simulink model "Drone"  (R2026a)
settings: Solver=VariableStepAuto  StopTime=500
undefined symbols (not defined in the file): magnitude
libraries: slpidlib x4, simulink_extras x1, sl3dlib x1, sim3dlib x1, uavsim3dlib x1
settings Model: Creator=siddharthreddy  LastModifiedBy=Sid

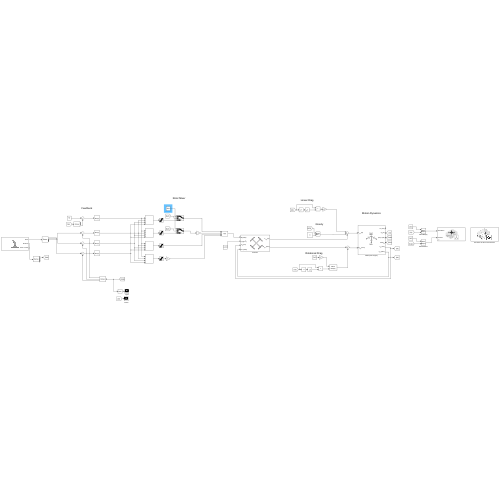
[thumbnail: Simulink's stored preview of the top-level diagram]
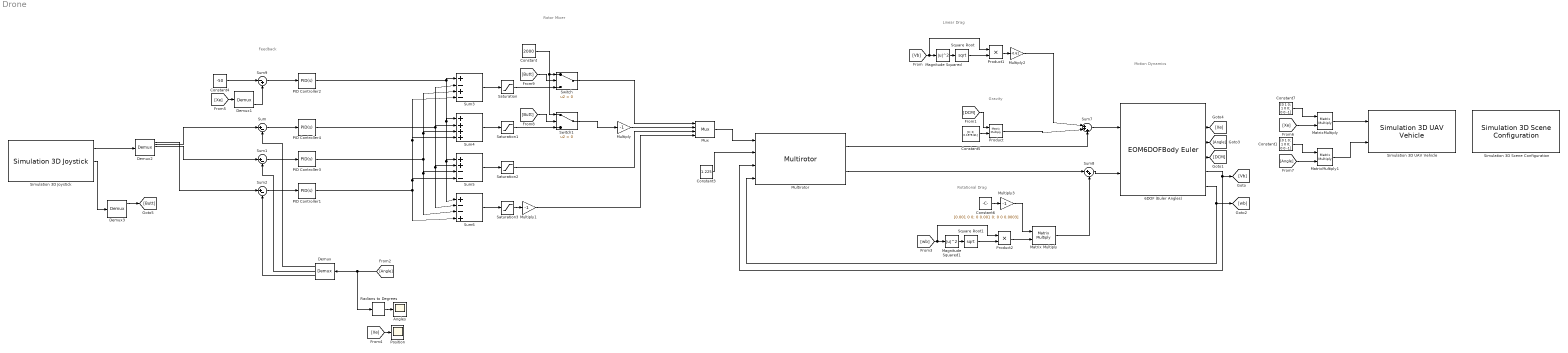
== system Drone ==
  note: Motion Dynamics
  note: Rotor Mixer
  note: Feedback
  note: Gravity
  note: Linear Drag
  note: Rotational Drag
  6DOF (Euler Angles) : EOM6DOFBodyEuler  xme_0=[0 0 -40]  eul_0=[.25 .25 .5]  mass_0=0.15  inertia=[0.0003 0 0; 0 0.0003 0; 0 0 0.0003]
  Angles : Scope
      settings: ActiveDisplayYMinimum=-79.706832912705636  ActiveDisplayYMaximum=125.45902835260904
  Constant : Constant  Value=2000
  Constant1 : Constant  Value=[0 1 0; 1 0 0; 0 0 -1]
  Constant3 : Constant  Value=1.225
  Constant4 : Constant  Value=-50
  Constant5 : Constant  Value=[0; 0; 0.15*9.81]
  Constant6 : Constant  Value=[0.001 0 0; 0 0.001 0; 0 0 0.0003]
  Constant7 : Constant  Value=[0 1 0; 1 0 0; 0 0 -1]
  Demux : Demux  Outputs=3
      settings: DisplayOption=none
  Demux1 : Demux  Outputs=3
      settings: DisplayOption=none
  Demux2 : Demux  Outputs=6
      settings: DisplayOption=none
  Demux3 : Demux  Outputs=8
      settings: DisplayOption=none
  Magnitude Squared : Math  Operator=magnitude^2
  Magnitude Squared1 : Math  Operator=magnitude^2
  Matrix Multiply : Product  Multiplication=Matrix(*)
  MatrixMultiply : Product  Multiplication=Matrix(*)
  MatrixMultiply1 : Product  Multiplication=Matrix(*)
  Multiply : Gain  Gain=-1
  Multiply1 : Gain  Gain=-1
  Multiply2 : Gain  Gain=-0.61
  Multiply3 : Gain  Gain=-1
  Multirotor : Multirotor  modelMode=With flap effects  armLength=0.06  rotorHeight=0  CT=0.08  CQ=0.001  radius=0.065/2
  Mux : Mux
  PID Controller1 : slpidlib/PID Controller  Controller=PID  Form=Parallel  TimeDomain=Continuous-time  UseExternalTs=off  SampleTime=-1  IntegratorMethod=Forward Euler  FilterMethod=Forward Euler  ControllerParametersSource=internal  P=1421.28268044684  I=470.589569781493  UseKiTs=off  D=956.469408662535  UseExternalDerivativeSource=off  N=11.7175649403718  UseFilter=on  TunerSelectOption=Transfer Function Based (PID Tuner App)  InitialConditionSource=internal  InitialConditionForIntegrator=0  InitialConditionForFilter=0  DifferentiatorICPrevScaledInput=0  ExternalReset=none  TrackingMode=off  Kt=1  LimitOutput=off  SatLimitsSource=internal  UpperSaturationLimit=inf  LowerSaturationLimit=-inf  LinearizeAsGain=on  AntiWindupMode=none  Kb=1  LimitIntegrator=off  UpperIntegratorSaturationLimit=inf  LowerIntegratorSaturationLimit=-inf  POutMin=[]  POutMax=[]  IOutMin=[]  IOutMax=[]  DOutMin=[]  DOutMax=[]  NOutMin=[]  NOutMax=[]  SumOutMin=[]  SumOutMax=[]  SaturationOutMin=[]  SaturationOutMax=[]  PParamMin=[]  PParamMax=[]  IParamMin=[]  IParamMax=[]  DParamMin=[]  DParamMax=[]  NParamMin=[]  NParamMax=[]  KbParamMin=[]  KbParamMax=[]  KtParamMin=[]  KtParamMax=[]  KbOutMin=[]  KbOutMax=[]  KtOutMin=[]  KtOutMax=[]  IntegratorOutMin=[]  IntegratorOutMax=[]  FilterOutMin=[]  FilterOutMax=[]  SumI1OutMin=[]  SumI1OutMax=[]  SumI2OutMin=[]  SumI2OutMax=[]  SumI3OutMin=[]  SumI3OutMax=[]  SumI4OutMin=[]  SumI4OutMax=[]  SumDOutMin=[]  SumDOutMax=[]  DifferentiatorOutMin=[]  DifferentiatorOutMax=[]  FilterDiffOutCoefMin=[]  FilterDiffOutCoefMax=[]  ReciprocalOutMin=[]  ReciprocalOutMax=[]  SumDenOutMin=[]  SumDenOutMax=[]  SumNumOutMin=[]  SumNumOutMax=[]  DivideOutMin=[]  DivideOutMax=[]  UdiffTsProdOutMin=[]  UdiffTsProdOutMax=[]  NTsProdOutMin=[]  NTsProdOutMax=[]  UintegralTsProdOutMin=[]  UintegralTsProdOutMax=[]  UngainTsProdOutMin=[]  UngainTsProdOutMax=[]  ClampingZeroOutDataTypeStr=Inherit: Inherit via back propagation  ClampingZeroOutMin=[]  ClampingZeroOutMax=[]  FilterDenConstantOutDataTypeStr=Inherit: Inherit via back propagation  FilterDenConstantOutMin=[]  FilterDenConstantOutMax=[]  PCopyOutDataTypeStr=Inherit: Inherit via back propagation  PCopyOutMin=[]  PCopyOutMax=[]  NCopyOutDataTypeStr=Inherit: Inherit via back propagation  NCopyOutMin=[]  NCopyOutMax=[]  IntegratorContinuousStateAttributes=''  IntegratorStateMustResolveToSignalObject=off  IntegratorRTWStateStorageClass=Auto  FilterContinuousStateAttributes=''  FilterStateMustResolveToSignalObject=off  FilterRTWStateStorageClass=Auto  ParallelPVariant=InternalParameters  IdealPVariant=Disabled  IVariant=InternalParameters  DVariant=InternalParameters  IntegratorVariant=Continuous  SatVariant=Disabled  AWVariant=Passthrough  PCopyVariant=Disabled  TRVariant=Disabled  FdbkBlocksVariant=Forward  IdealPFdbkVariant=Disabled  SatFdbkVariant=Disabled  DerivativeFilterVariant=ContFilter  NVariant=InternalParameters  NCopyVariant=Disabled  FilterICVariant=InternalICsFilter  IntegratorICVariant=InternalICs  ExternalResetVariant=Disabled  TRSumVariant=Passthrough  SumFdbkVariant=Disabled  SumVariant=Sum_PID  TsampFilterVariant=InternalTs  TsampNgainVariant=Passthrough  TsampIntegralVariant=Disabled_SignalSpec  ExternalSaturationOutDataTypeStr=Inherit: Same as second input  DerivativeSourceVariant=ErrorSignal  PreIntVariant=InternalPreInt
  PID Controller2 : slpidlib/PID Controller  Controller=PID  Form=Parallel  TimeDomain=Continuous-time  UseExternalTs=off  SampleTime=-1  IntegratorMethod=Forward Euler  FilterMethod=Forward Euler  ControllerParametersSource=internal  P=465.549469406637  I=214.212668672937  UseKiTs=off  D=189.884905448547  UseExternalDerivativeSource=off  N=1142.8279760416  UseFilter=on  TunerSelectOption=Transfer Function Based (PID Tuner App)  InitialConditionSource=internal  InitialConditionForIntegrator=0  InitialConditionForFilter=0  DifferentiatorICPrevScaledInput=0  ExternalReset=none  TrackingMode=off  Kt=1  LimitOutput=off  SatLimitsSource=internal  UpperSaturationLimit=inf  LowerSaturationLimit=-inf  LinearizeAsGain=on  AntiWindupMode=none  Kb=1  LimitIntegrator=off  UpperIntegratorSaturationLimit=inf  LowerIntegratorSaturationLimit=-inf  POutMin=[]  POutMax=[]  IOutMin=[]  IOutMax=[]  DOutMin=[]  DOutMax=[]  NOutMin=[]  NOutMax=[]  SumOutMin=[]  SumOutMax=[]  SaturationOutMin=[]  SaturationOutMax=[]  PParamMin=[]  PParamMax=[]  IParamMin=[]  IParamMax=[]  DParamMin=[]  DParamMax=[]  NParamMin=[]  NParamMax=[]  KbParamMin=[]  KbParamMax=[]  KtParamMin=[]  KtParamMax=[]  KbOutMin=[]  KbOutMax=[]  KtOutMin=[]  KtOutMax=[]  IntegratorOutMin=[]  IntegratorOutMax=[]  FilterOutMin=[]  FilterOutMax=[]  SumI1OutMin=[]  SumI1OutMax=[]  SumI2OutMin=[]  SumI2OutMax=[]  SumI3OutMin=[]  SumI3OutMax=[]  SumI4OutMin=[]  SumI4OutMax=[]  SumDOutMin=[]  SumDOutMax=[]  DifferentiatorOutMin=[]  DifferentiatorOutMax=[]  FilterDiffOutCoefMin=[]  FilterDiffOutCoefMax=[]  ReciprocalOutMin=[]  ReciprocalOutMax=[]  SumDenOutMin=[]  SumDenOutMax=[]  SumNumOutMin=[]  SumNumOutMax=[]  DivideOutMin=[]  DivideOutMax=[]  UdiffTsProdOutMin=[]  UdiffTsProdOutMax=[]  NTsProdOutMin=[]  NTsProdOutMax=[]  UintegralTsProdOutMin=[]  UintegralTsProdOutMax=[]  UngainTsProdOutMin=[]  UngainTsProdOutMax=[]  ClampingZeroOutDataTypeStr=Inherit: Inherit via back propagation  ClampingZeroOutMin=[]  ClampingZeroOutMax=[]  FilterDenConstantOutDataTypeStr=Inherit: Inherit via back propagation  FilterDenConstantOutMin=[]  FilterDenConstantOutMax=[]  PCopyOutDataTypeStr=Inherit: Inherit via back propagation  PCopyOutMin=[]  PCopyOutMax=[]  NCopyOutDataTypeStr=Inherit: Inherit via back propagation  NCopyOutMin=[]  NCopyOutMax=[]  IntegratorContinuousStateAttributes=''  IntegratorStateMustResolveToSignalObject=off  IntegratorRTWStateStorageClass=Auto  FilterContinuousStateAttributes=''  FilterStateMustResolveToSignalObject=off  FilterRTWStateStorageClass=Auto  ParallelPVariant=InternalParameters  IdealPVariant=Disabled  IVariant=InternalParameters  DVariant=InternalParameters  IntegratorVariant=Continuous  SatVariant=Disabled  AWVariant=Passthrough  PCopyVariant=Disabled  TRVariant=Disabled  FdbkBlocksVariant=Forward  IdealPFdbkVariant=Disabled  SatFdbkVariant=Disabled  DerivativeFilterVariant=ContFilter  NVariant=InternalParameters  NCopyVariant=Disabled  FilterICVariant=InternalICsFilter  IntegratorICVariant=InternalICs  ExternalResetVariant=Disabled  TRSumVariant=Passthrough  SumFdbkVariant=Disabled  SumVariant=Sum_PID  TsampFilterVariant=InternalTs  TsampNgainVariant=Passthrough  TsampIntegralVariant=Disabled_SignalSpec  ExternalSaturationOutDataTypeStr=Inherit: Same as second input  DerivativeSourceVariant=ErrorSignal  PreIntVariant=InternalPreInt
  PID Controller3 : slpidlib/PID Controller  Controller=PID  Form=Parallel  TimeDomain=Continuous-time  UseExternalTs=off  SampleTime=-1  IntegratorMethod=Forward Euler  FilterMethod=Forward Euler  ControllerParametersSource=internal  P=1.53294785605493  I=0.217782758826352  UseKiTs=off  D=2.68640511728312  UseExternalDerivativeSource=off  N=361.393937805181  UseFilter=on  TunerSelectOption=Transfer Function Based (PID Tuner App)  InitialConditionSource=internal  InitialConditionForIntegrator=0  InitialConditionForFilter=0  DifferentiatorICPrevScaledInput=0  ExternalReset=none  TrackingMode=off  Kt=1  LimitOutput=off  SatLimitsSource=internal  UpperSaturationLimit=inf  LowerSaturationLimit=-inf  LinearizeAsGain=on  AntiWindupMode=none  Kb=1  LimitIntegrator=off  UpperIntegratorSaturationLimit=inf  LowerIntegratorSaturationLimit=-inf  POutMin=[]  POutMax=[]  IOutMin=[]  IOutMax=[]  DOutMin=[]  DOutMax=[]  NOutMin=[]  NOutMax=[]  SumOutMin=[]  SumOutMax=[]  SaturationOutMin=[]  SaturationOutMax=[]  PParamMin=[]  PParamMax=[]  IParamMin=[]  IParamMax=[]  DParamMin=[]  DParamMax=[]  NParamMin=[]  NParamMax=[]  KbParamMin=[]  KbParamMax=[]  KtParamMin=[]  KtParamMax=[]  KbOutMin=[]  KbOutMax=[]  KtOutMin=[]  KtOutMax=[]  IntegratorOutMin=[]  IntegratorOutMax=[]  FilterOutMin=[]  FilterOutMax=[]  SumI1OutMin=[]  SumI1OutMax=[]  SumI2OutMin=[]  SumI2OutMax=[]  SumI3OutMin=[]  SumI3OutMax=[]  SumI4OutMin=[]  SumI4OutMax=[]  SumDOutMin=[]  SumDOutMax=[]  DifferentiatorOutMin=[]  DifferentiatorOutMax=[]  FilterDiffOutCoefMin=[]  FilterDiffOutCoefMax=[]  ReciprocalOutMin=[]  ReciprocalOutMax=[]  SumDenOutMin=[]  SumDenOutMax=[]  SumNumOutMin=[]  SumNumOutMax=[]  DivideOutMin=[]  DivideOutMax=[]  UdiffTsProdOutMin=[]  UdiffTsProdOutMax=[]  NTsProdOutMin=[]  NTsProdOutMax=[]  UintegralTsProdOutMin=[]  UintegralTsProdOutMax=[]  UngainTsProdOutMin=[]  UngainTsProdOutMax=[]  ClampingZeroOutDataTypeStr=Inherit: Inherit via back propagation  ClampingZeroOutMin=[]  ClampingZeroOutMax=[]  FilterDenConstantOutDataTypeStr=Inherit: Inherit via back propagation  FilterDenConstantOutMin=[]  FilterDenConstantOutMax=[]  PCopyOutDataTypeStr=Inherit: Inherit via back propagation  PCopyOutMin=[]  PCopyOutMax=[]  NCopyOutDataTypeStr=Inherit: Inherit via back propagation  NCopyOutMin=[]  NCopyOutMax=[]  IntegratorContinuousStateAttributes=''  IntegratorStateMustResolveToSignalObject=off  IntegratorRTWStateStorageClass=Auto  FilterContinuousStateAttributes=''  FilterStateMustResolveToSignalObject=off  FilterRTWStateStorageClass=Auto  ParallelPVariant=InternalParameters  IdealPVariant=Disabled  IVariant=InternalParameters  DVariant=InternalParameters  IntegratorVariant=Continuous  SatVariant=Disabled  AWVariant=Passthrough  PCopyVariant=Disabled  TRVariant=Disabled  FdbkBlocksVariant=Forward  IdealPFdbkVariant=Disabled  SatFdbkVariant=Disabled  DerivativeFilterVariant=ContFilter  NVariant=InternalParameters  NCopyVariant=Disabled  FilterICVariant=InternalICsFilter  IntegratorICVariant=InternalICs  ExternalResetVariant=Disabled  TRSumVariant=Passthrough  SumFdbkVariant=Disabled  SumVariant=Sum_PID  TsampFilterVariant=InternalTs  TsampNgainVariant=Passthrough  TsampIntegralVariant=Disabled_SignalSpec  ExternalSaturationOutDataTypeStr=Inherit: Same as second input  DerivativeSourceVariant=ErrorSignal  PreIntVariant=InternalPreInt
  PID Controller4 : slpidlib/PID Controller  Controller=PID  Form=Parallel  TimeDomain=Continuous-time  UseExternalTs=off  SampleTime=-1  IntegratorMethod=Forward Euler  FilterMethod=Forward Euler  ControllerParametersSource=internal  P=-1.53294785605493  I=-0.217782758826352  UseKiTs=off  D=-2.68640511728312  UseExternalDerivativeSource=off  N=361.393937805181  UseFilter=on  TunerSelectOption=Transfer Function Based (PID Tuner App)  InitialConditionSource=internal  InitialConditionForIntegrator=0  InitialConditionForFilter=0  DifferentiatorICPrevScaledInput=0  ExternalReset=none  TrackingMode=off  Kt=1  LimitOutput=off  SatLimitsSource=internal  UpperSaturationLimit=inf  LowerSaturationLimit=-inf  LinearizeAsGain=on  AntiWindupMode=none  Kb=1  LimitIntegrator=off  UpperIntegratorSaturationLimit=inf  LowerIntegratorSaturationLimit=-inf  POutMin=[]  POutMax=[]  IOutMin=[]  IOutMax=[]  DOutMin=[]  DOutMax=[]  NOutMin=[]  NOutMax=[]  SumOutMin=[]  SumOutMax=[]  SaturationOutMin=[]  SaturationOutMax=[]  PParamMin=[]  PParamMax=[]  IParamMin=[]  IParamMax=[]  DParamMin=[]  DParamMax=[]  NParamMin=[]  NParamMax=[]  KbParamMin=[]  KbParamMax=[]  KtParamMin=[]  KtParamMax=[]  KbOutMin=[]  KbOutMax=[]  KtOutMin=[]  KtOutMax=[]  IntegratorOutMin=[]  IntegratorOutMax=[]  FilterOutMin=[]  FilterOutMax=[]  SumI1OutMin=[]  SumI1OutMax=[]  SumI2OutMin=[]  SumI2OutMax=[]  SumI3OutMin=[]  SumI3OutMax=[]  SumI4OutMin=[]  SumI4OutMax=[]  SumDOutMin=[]  SumDOutMax=[]  DifferentiatorOutMin=[]  DifferentiatorOutMax=[]  FilterDiffOutCoefMin=[]  FilterDiffOutCoefMax=[]  ReciprocalOutMin=[]  ReciprocalOutMax=[]  SumDenOutMin=[]  SumDenOutMax=[]  SumNumOutMin=[]  SumNumOutMax=[]  DivideOutMin=[]  DivideOutMax=[]  UdiffTsProdOutMin=[]  UdiffTsProdOutMax=[]  NTsProdOutMin=[]  NTsProdOutMax=[]  UintegralTsProdOutMin=[]  UintegralTsProdOutMax=[]  UngainTsProdOutMin=[]  UngainTsProdOutMax=[]  ClampingZeroOutDataTypeStr=Inherit: Inherit via back propagation  ClampingZeroOutMin=[]  ClampingZeroOutMax=[]  FilterDenConstantOutDataTypeStr=Inherit: Inherit via back propagation  FilterDenConstantOutMin=[]  FilterDenConstantOutMax=[]  PCopyOutDataTypeStr=Inherit: Inherit via back propagation  PCopyOutMin=[]  PCopyOutMax=[]  NCopyOutDataTypeStr=Inherit: Inherit via back propagation  NCopyOutMin=[]  NCopyOutMax=[]  IntegratorContinuousStateAttributes=''  IntegratorStateMustResolveToSignalObject=off  IntegratorRTWStateStorageClass=Auto  FilterContinuousStateAttributes=''  FilterStateMustResolveToSignalObject=off  FilterRTWStateStorageClass=Auto  ParallelPVariant=InternalParameters  IdealPVariant=Disabled  IVariant=InternalParameters  DVariant=InternalParameters  IntegratorVariant=Continuous  SatVariant=Disabled  AWVariant=Passthrough  PCopyVariant=Disabled  TRVariant=Disabled  FdbkBlocksVariant=Forward  IdealPFdbkVariant=Disabled  SatFdbkVariant=Disabled  DerivativeFilterVariant=ContFilter  NVariant=InternalParameters  NCopyVariant=Disabled  FilterICVariant=InternalICsFilter  IntegratorICVariant=InternalICs  ExternalResetVariant=Disabled  TRSumVariant=Passthrough  SumFdbkVariant=Disabled  SumVariant=Sum_PID  TsampFilterVariant=InternalTs  TsampNgainVariant=Passthrough  TsampIntegralVariant=Disabled_SignalSpec  ExternalSaturationOutDataTypeStr=Inherit: Same as second input  DerivativeSourceVariant=ErrorSignal  PreIntVariant=InternalPreInt
  Position : Scope
      settings: ActiveDisplayYMinimum=-335.35566969073909  ActiveDisplayYMaximum=208.27591374665826
  Product : Product  Multiplication=Matrix(*)
  Product1 : Product
  Product2 : Product
  Radians to Degrees : simulink_extras/Transformations/Radians to Degrees
  Saturation{,1..3} (4 alike) : Saturate  UpperLimit=3000  LowerLimit=0
  Simulation 3D Joystick : sl3dlib/Simulation 3D/Hardware Interface/Simulation 3D Joystick  joyid=1  adjustports=on  forcefeed=off
  Simulation 3D Scene Configuration : sim3dlib/Simulation 3D Scene Configuration  Priority=0  ProjectFormat=Default Scenes  SceneDesc=US city block  ProjectName=C:\Program Files\MATLAB\R2026a\toolbox\shared\sim3d_projects\automotive_project_windows\UE\WindowsNoEditor\VehicleSimulation.exe  ScenePath=/Game/Maps/USCityBlock  EnableOpenDRIVE=off  vehTagList={'Custom';'Scene Origin';'SimulinkVehicle1'}  vehTag=SimulinkVehicle1  AttachedCameraRelativeTranslation=[0 0 0]  FreeCameraDefaultInitialTranslation=[-6, 0, 2]  AttachedCameraRelativeRotation=[0, -15, 0]  FreeCameraDefaultInitialRotation=[0, -15, 0]  ViewpointName=Custom  FreeCameraInitialTranslation=[0, 0, 0]  FreeCameraInitialRotation=[0, 0, 0]  OpVisEn=off  Ts=1/60  EnableWindow=on  EnableRemoteAccess=off  SimulationMode=CoSimulation  SimulateUsing=Interpreted execution  EnableAnimationRecording=off  OverrideDefaultRecording=off  AnimationRecordingFileName=sim3dAnimation.mat  AnimationRecordingInterval=[0 inf]  EnableWeather=off  SunAzimuth=90  SunAltitude=40.0  EnableGeospatialSun=off  Latitude=0  Longitude=0  Date=2023-01-01  Time=10:30:00  GeoTimeZone=-5.0  SunDaylightSaving=off  wind=1  clouds=10  EnableVolumetricClouds=off  CloudCoverage=0  CloudAltitude=6  fog=0  rain=0  RaindropsEffect=off  SnowDensity=0  EnableGeospatial=off  TilesetSource=Earth terrain  UseTrueOrigin=off  OriginHeight=200  OriginLatitude=40.744652  OriginLongitude=-73.988864  MapStyle=Aerial  AdditionalAssetIDs=[]  UseAdvancedSunSky=off  SolarTime=11  TimeZone=-5  Day=21  Month=9  Year=2022  UseDaylightSavingTime=on  DSTStartDay=10  DSTStartMonth=3  DSTEndDay=3  DSTEndMonth=11  DSTSwitchHour=2  sensorTag=MainCamera1  sensorId=1  sensorName=MainCamera1  mountLoc=Origin  offsetFlag=off  tmountOffset=[0, 0, 0]  rmountOffset=[0, 0, 0]  HorizontalResolution=1280  VerticalResolution=720  HorizontalFOV=60  mountPoint=[0 0 0]  mountOrientation=[0 0 0]  aMode=4  ID=1  GeoTrigger=Inactive  ViewNameList={'Custom'}  ViewTranslationList={'[0 0 0]'}  ViewRotationList={'[0 0 0]'}
      settings: LibrarySourceBlock=uavsim3dlib/Simulation 3D Scene Configuration
  Simulation 3D UAV Vehicle : uavsim3dlib/Simulation 3D UAV Vehicle  Priority=-1  Mesh=Quadrotor  MeshPath=/MathWorksUAVContent/UAVs/HexaRotorUAV/HexaRotor.HexaRotor  Color=Black  ActorName=SimulinkVehicle1  UseGlobalFrame=off  InitialTranslation=[0 0 0]  InitialRotation=[0 0 0]  InitialTranslationGlobal=[0 0 0]  InitialGeoOrigin=[0 0 0]  InitialRotationGlobal=[0 0 0]  SampleTime=-1  ActorType=SimulinkVehicle  ID=1  aMode=4  ActorTag=SimulinkVehicle1
  Square Root : Sqrt
  Square Root1 : Sqrt
  Sum : Sum  Inputs=|+-
  Sum1 : Sum  Inputs=|+-
  Sum2 : Sum  Inputs=|+-
  Sum3 : Sum  Inputs=|+-+-
  Sum4 : Sum  Inputs=|++++
  Sum5 : Sum  Inputs=|++--
  Sum6 : Sum  Inputs=|+--+
  Sum7 : Sum  Inputs=|+++
  Sum8 : Sum  Inputs=|++
  Sum9 : Sum  Inputs=|-+
  Switch : Switch  Criteria=u2 > Threshold  SaturateOnIntegerOverflow=off  InputSameDT=off
  Switch1 : Switch  Criteria=u2 > Threshold  SaturateOnIntegerOverflow=off  InputSameDT=off
  wires:
  Sum/1 -> PID Controller4/1
  Sum2/1 -> PID Controller1/1
  Demux/1 -> Sum/2
  Demux/2 -> Sum1/2
  Demux/3 -> Sum2/2
  PID Controller1/1 -> Sum6/4, Sum3/4, Sum4/4, Sum5/4
  PID Controller3/1 -> Sum6/3, Sum5/3, Sum3/3, Sum4/3
  PID Controller4/1 -> Sum3/2, Sum4/2, Sum6/2, Sum5/2
  Mux/1 -> Multirotor/1
  Constant3/1 -> Multirotor/2
  PID Controller2/1 -> Sum4/1, Sum5/1, Sum6/1, Sum3/1
  Sum1/1 -> PID Controller3/1
  Sum3/1 -> Saturation/1
  Sum4/1 -> Saturation1/1
  Sum5/1 -> Saturation2/1
  Sum6/1 -> Saturation3/1
  Radians to Degrees/1 -> Angles/1
  Saturation2/1 -> Mux/3
  Saturation3/1 -> Multiply1/1
  Multiply/1 -> Mux/2
  Multiply1/1 -> Mux/4
  Magnitude Squared/1 -> Square Root/1
  Product1/1 -> Multiply2/1
  [Vb] -> Product1/1, Magnitude Squared/1
  6DOF (Euler Angles)/4 -> [DCM]
  Square Root/1 -> Product1/2
  6DOF (Euler Angles)/5 -> [Vb], Multirotor/3
  6DOF (Euler Angles)/6 -> [wb], Multirotor/4
  [DCM] -> Product/1
  Constant5/1 -> Product/2
  Multirotor/1 -> Sum7/3
  Multiply2/1 -> Sum7/1
  Sum7/1 -> 6DOF (Euler Angles)/1
  6DOF (Euler Angles)/3 -> [Angle]
  [Angle] -> Radians to Degrees/1, Demux/1
  Product/1 -> Sum7/2
  Product2/1 -> Matrix Multiply/2
  [wb] -> Product2/1, Magnitude Squared1/1
  Magnitude Squared1/1 -> Square Root1/1
  Square Root1/1 -> Product2/2
  Constant6/1 -> Multiply3/1
  Multiply3/1 -> Matrix Multiply/1
  Matrix Multiply/1 -> Sum8/2
  Sum8/1 -> 6DOF (Euler Angles)/2
  Multirotor/2 -> Sum8/1
  6DOF (Euler Angles)/2 -> [Xe]
  [Xe] -> Position/1
  Constant4/1 -> Sum9/1
  Sum9/1 -> PID Controller2/1
  Demux1/3 -> Sum9/2
  [Xe] -> Demux1/1
  Constant7/1 -> MatrixMultiply/1
  [Xe] -> MatrixMultiply/2
  MatrixMultiply/1 -> Simulation 3D UAV Vehicle/1
  Simulation 3D Joystick/1 -> Demux2/1
  [Angle] -> MatrixMultiply1/2
  Constant1/1 -> MatrixMultiply1/1
  MatrixMultiply1/1 -> Simulation 3D UAV Vehicle/2
  Simulation 3D Joystick/2 -> Demux3/1
  Demux2/2 -> Sum/1
  Demux2/3 -> Sum1/1
  Demux2/1 -> Sum2/1
  Switch/1 -> Mux/1
  Switch1/1 -> Multiply/1
  Saturation/1 -> Switch/3
  Saturation1/1 -> Switch1/3
  [Butt] -> Switch/2
  [Butt] -> Switch1/2
  Constant/1 -> Switch/1, Switch1/1
  Demux3/2 -> [Butt]
